simulink model "lab56"  (R2025b)
settings: Solver=VariableStepAuto  StartTime=0.0  StopTime=10.0  RelTol=1e-3
undefined symbols (not defined in the file): A, Bss, C, Css, Dss, K, Lw, x0, xhat0
libraries: simulink x3
settings Model: Creator=Nickolay  LastModifiedBy=Nickolay

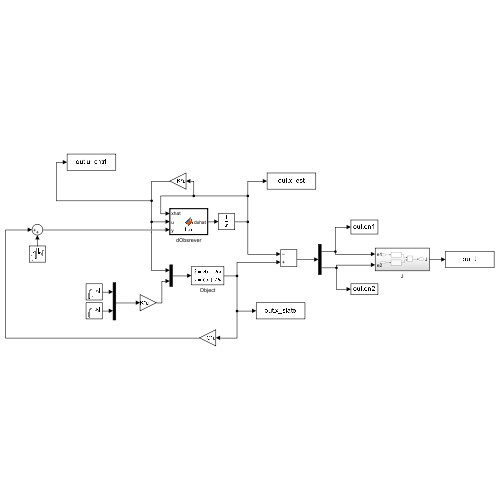
[thumbnail: Simulink's stored preview of the top-level diagram]
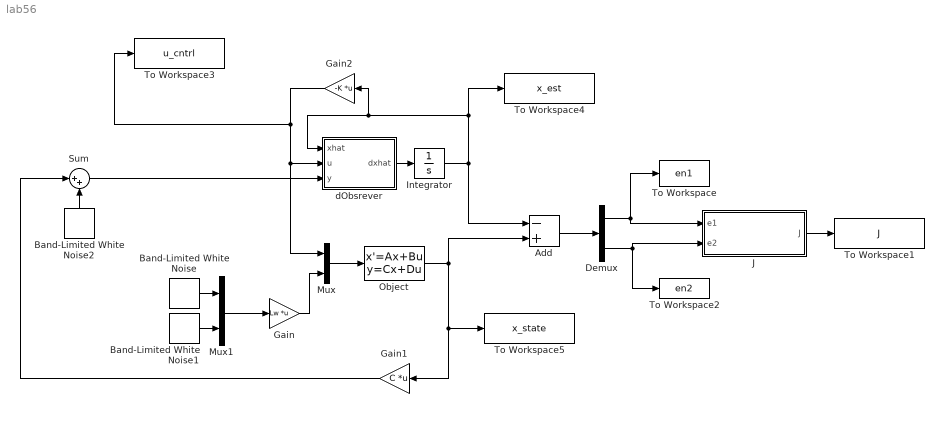
== system lab56 ==
  Add : Sum  Inputs=-+
  Band-Limited White Noise : simulink/Sources/Band-Limited White Noise  Cov=1  Ts=0.001  seed=seedW1
  Band-Limited White Noise1 : simulink/Sources/Band-Limited White Noise  Cov=1  Ts=0.001  seed=seedW2
  Band-Limited White Noise2 : simulink/Sources/Band-Limited White Noise  Cov=V  Ts=0.001  seed=seedV
  Demux : Demux  Outputs=2
  Gain : Gain  Gain=Lw  Multiplication=Matrix(K*u)
  Gain1 : Gain  Gain=C  Multiplication=Matrix(K*u)
  Gain2 : Gain  Gain=-K  Multiplication=Matrix(K*u)
  Integrator : Integrator  InitialCondition=xhat0
  J : Subsystem
  Mux : Mux  Inputs=2
  Mux1 : Mux  Inputs=2
  Object : StateSpace  A=A  B=Bss  C=Css  D=Dss  InitialCondition=x0
  Sum : Sum  Inputs=|++
  To Workspace : ToWorkspace  VariableName=en1  SaveFormat=Timeseries  SampleTime=-1
  To Workspace1 : ToWorkspace  VariableName=J  SaveFormat=Timeseries  SampleTime=-1
  To Workspace2 : ToWorkspace  VariableName=en2  SaveFormat=Timeseries  SampleTime=-1
  To Workspace3 : ToWorkspace  VariableName=u_cntrl  SaveFormat=Timeseries  SampleTime=-1
  To Workspace4 : ToWorkspace  VariableName=x_est  SaveFormat=Timeseries  SampleTime=-1
  To Workspace5 : ToWorkspace  VariableName=x_state  SaveFormat=Timeseries  SampleTime=-1
  dObsrever : MATLAB Function  TreatAsAtomicUnit=on
  wires:
  Mux/1 -> Object/1
  Gain2/1 -> dObsrever/2(u), Mux/1, To Workspace3/1
  Band-Limited White Noise/1 -> Mux1/1
  Band-Limited White Noise1/1 -> Mux1/2
  Mux1/1 -> Gain/1
  Gain/1 -> Mux/2
  dObsrever/1(dxhat) -> Integrator/1
  Object/1 -> To Workspace5/1, Gain1/1, Add/2
  Integrator/1 -> To Workspace4/1, dObsrever/1(xhat), Gain2/1, Add/1
  Add/1 -> Demux/1
  Demux/1 -> To Workspace/1, J/1(e1)
  Demux/2 -> J/2(e2), To Workspace2/1
  J/1(J) -> To Workspace1/1
  Gain1/1 -> Sum/1
  Band-Limited White Noise2/1 -> Sum/2
  Sum/1 -> dObsrever/3(y)

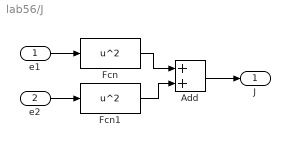
== system lab56/J ==
  e1 : Inport
  e2 : Inport  Port=2
  Add : Sum
  Fcn : Fcn  Expr=u^2
  Fcn1 : Fcn  Expr=u^2
  J : Outport
  wires:
  e2/1 -> Fcn1/1
  e1/1 -> Fcn/1
  Fcn/1 -> Add/1
  Fcn1/1 -> Add/2
  Add/1 -> J/1

== matlab function lab56/dObsrever ==
  data: xhat input; u input; dxhat output; y input
function dxhat = fcn(xhat, u, y)

A = [0 1; -9 -2];
B = [8; 4];
C = [1 0];
L = [0.657670; -0.658735];

dxhat = A*xhat + B*u + L*(y - C*xhat);

end
